simulink library "three_phase_voltage_emulator_mfcn"  (R2026a)
settings: Solver=VariableStepAuto
settings Model: Creator=pwr-control  LastModifiedBy=pwr-control

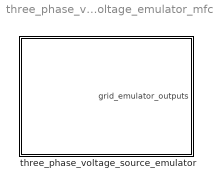
== system three_phase_voltage_emulator_mfcn ==
  three_phase_voltage_source_emulator : Subsystem  mask(Three-phase voltage emulator (MATLAB Function)){freq=50, ugrid_nom=690, vp_xi_pu=1, vp_eta_pu=0, vn_xi_pu=0, vn_eta_pu=0, fcut_lvrt=50}
      mask prompts: freq "Nominal Frequency [Hz]"; ugrid_nom "Nominal Voltage [V]"; vp_xi_pu "vp_xi_pu [pu]"; vp_eta_pu "vp_eta_pu [pu]"; vn_xi_pu "vn_xi_pu [pu]"; vn_eta_pu "vn_eta_pu [pu]"; fcut_lvrt "LVRT_flt_ss [Hz]"
      mask help:
      | Copy of three_phase_voltage_emulator/three_phase_voltage_source_emulator written as one MATLAB Function block: same parameters, same output bus grid_emulator_outputs (ua_grid_emu, ub_grid_emu, uc_grid_emu, gamma_grid_emulator, omega_grid_emulator).
      |
      | The grid angle and the first-order LVRT filters are written in closed form as functions of the simulation time, so the block has no states and 3 non-virtual blocks (the original has 44). The simulation must start at t = 0.
      mask Help: web('https://github.com/pwr-control/library/blob/dev/library/masked_models/power_supply_emulators/README.md', '-browser')
      mask Display:
      | disp(sprintf('three-phase voltage\nemulator\nMATLAB Function'))
      | port_label('output', 1, 'grid_emulator_outputs')

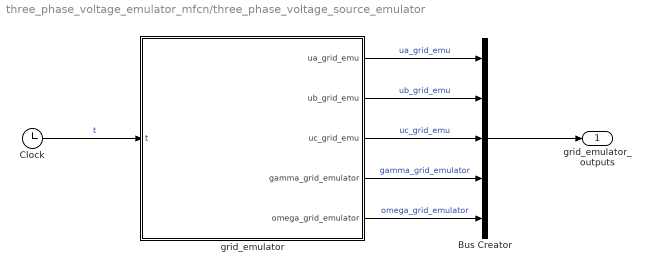
== system three_phase_voltage_emulator_mfcn/three_phase_voltage_source_emulator ==
  Clock : Clock
  grid_emulator : MATLAB Function  TreatAsAtomicUnit=on
  Bus Creator : BusCreator  Inputs=5
  grid_emulator_outputs : Outport  VectorParamsAs1DForOutWhenUnconnected=off
  wires:
  Clock/1 -> grid_emulator/1(t)  "t"
  grid_emulator/1(ua_grid_emu) -> Bus Creator/1  "ua_grid_emu"
  grid_emulator/2(ub_grid_emu) -> Bus Creator/2  "ub_grid_emu"
  grid_emulator/3(uc_grid_emu) -> Bus Creator/3  "uc_grid_emu"
  grid_emulator/4(gamma_grid_emulator) -> Bus Creator/4  "gamma_grid_emulator"
  grid_emulator/5(omega_grid_emulator) -> Bus Creator/5  "omega_grid_emulator"
  Bus Creator/1 -> grid_emulator_outputs/1

== matlab function three_phase_voltage_emulator_mfcn/three_phase_voltage_source_emulator/grid_emulator ==
  data: t input; ua_grid_emu output; ub_grid_emu output; uc_grid_emu output; gamma_grid_emulator output; omega_grid_emulator output; freq parameter; ugrid_nom parameter; vp_xi_pu parameter; vp_eta_pu parameter; vn_xi_pu parameter; vn_eta_pu parameter; fcut_lvrt parameter
function [ua_grid_emu, ub_grid_emu, uc_grid_emu, gamma_grid_emulator, omega_grid_emulator] = grid_emulator(t, ...
    freq, ugrid_nom, vp_xi_pu, vp_eta_pu, vn_xi_pu, vn_eta_pu, fcut_lvrt)
%#codegen
% GRID_EMULATOR
% MATLAB Function copy of three_phase_voltage_emulator/three_phase_voltage_source_emulator:
% same mask parameters, same output bus. The original integrates five continuous states
% (the grid angle and four first-order LVRT filters fed by constants). Their solution is
% known in closed form, so here it is written as a function of the time t and the block
% has no states.
%
% INPUT
%   t : simulation time [s], from the Clock block (the simulation must start at t = 0,
%       where the states of the original start from zero)
%
% PARAMETERS (mask parameters of the block: arguments with scope Parameter, no ports)
%   freq      : nominal frequency [Hz]
%   ugrid_nom : nominal line-to-line rms voltage [V]
%   vp_xi_pu, vp_eta_pu, vn_xi_pu, vn_eta_pu : positive / negative sequence references [pu]
%   fcut_lvrt : cut-off frequency of the first-order LVRT filter [Hz]
%
% OUTPUTS (elements of the bus grid_emulator_outputs, same order as the original)
%   ua_grid_emu, ub_grid_emu, uc_grid_emu : phase voltages [V]
%   gamma_grid_emulator : grid angle, wrapped to [-pi, pi) [rad]
%   omega_grid_emulator : grid angular frequency [rad/s]

% phase_gen: Constant omega_grid_emulator_nom -> Integrator (starts from 0) -> bounder
omega_grid_emulator = freq*2*pi;
gamma_grid_emulator = -pi + mod(omega_grid_emulator*t + 3*pi, 2*pi);

% sequences_voltage_source: Constant -> LVRT_ss_flt -> Gain ugrid_phase.
% LVRT_ss_flt is 1/(s/(2*pi*fcut_lvrt) + 1) with zero initial state: with a constant
% input u applied from t = 0 its output is (1 - exp(-2*pi*fcut_lvrt*t))*u.
k_flt = 0;
if t > 0
    k_flt = 1 - exp(-2*pi*fcut_lvrt*t);
end
ugrid_phase = ugrid_nom/sqrt(3/2);
vp_xi  = ugrid_phase*(k_flt*vp_xi_pu);
vp_eta = ugrid_phase*(k_flt*vp_eta_pu);
vn_xi  = ugrid_phase*(k_flt*vn_xi_pu);
vn_eta = ugrid_phase*(k_flt*vn_eta_pu);

% voltage_reference: xieta2alphabeta_pos + xieta2alphabeta_neg -> alphabeta2abc
c = cos(gamma_grid_emulator);
s = sin(gamma_grid_emulator);
alpha = (vp_xi*c - vp_eta*s) + (vn_xi*c + vn_eta*s);
beta  = (vp_xi*s + vp_eta*c) + (-vn_xi*s + vn_eta*c);

ua_grid_emu = alpha;
ub_grid_emu = -0.5*alpha + sqrt(3)/2*beta;
uc_grid_emu = -0.5*alpha - sqrt(3)/2*beta;
end
